simulink model "GuidanceLaw"  (R2023b)
settings: Solver=ode4  StartTime=0.0  StopTime=400  FixedStep=0.05  RelTol=1e-3
values from neighbouring files (symbols this model uses):
  APCMD_TYPE : value not decoded    [apDataDictionary.sldd]
  missionRoutePlan_struct = struct(      'validWpNum_u8', uint8(5),      'missionRoute_struct', repmat(wpDefault_struct, double(maxWpNum_u8), 1))    [initMissionRoutePlan_MC.m]
  MSSN_TYPE : value not decoded    [apDataDictionary.sldd]
  setPoint_struct = struct('lat_deg_d',double(31.200000),'lon_deg_d',double(121.500000),'alt_m_f',single(100),'yaw_deg_f',single(0))    [APTest.m]
undefined symbols (not defined in the file or in its folder): apParams
libraries: simulink x13, simulink_extras x3
(part 6 of 7)

== stateflow chart GuidanceLaw/Subsystem/TaskModeManager ==
  note: tryBwdTiltPlan函数完成其他条件的达成，包括规划是否成功
  state AUTO_BACKWARD_TILT
    entry:
    routeUpdate_b=candidateRouteUpdate_b;
    mssnType_u8=MSSN_TYPE.AUTO_BACKWARD_TILT;
    validWpNum_u8=candidateValidWpNum_u8;
    route_struct=candidateRoute_struct;
    during:
    routeUpdate_b=false;
  note: tryFwdTiltPlan函数完成其他条件的达成，包括规划是否成功
  state AUTO_FORWARD_TILT
    entry:
    routeUpdate_b=candidateRouteUpdate_b;
    mssnType_u8=MSSN_TYPE.AUTO_FORWARD_TILT;
    validWpNum_u8=candidateValidWpNum_u8;
    route_struct=candidateRoute_struct;
    during:
    routeUpdate_b=false;
  state ATT_EMERGENCY_LAND
    entry:
    routeUpdate_b=candidateRouteUpdate_b;
    mssnType_u8=mssnTypePre_u8;
    validWpNum_u8=candidateValidWpNum_u8;
    route_struct=candidateRoute_struct;
    during:
    routeUpdate_b=false;
  state IDLE
    entry:
    routeUpdate_b=false;
    mssnType_u8=MSSN_TYPE.IDLE;
    validWpNum_u8=uint8(0);
    route_struct=GenerateDefaultRoute();
  state RTH
    entry:
    routeUpdate_b=candidateRouteUpdate_b;
    mssnType_u8=MSSN_TYPE.RTH;
    validWpNum_u8=candidateValidWpNum_u8;
    route_struct=candidateRoute_struct;
    during:
    routeUpdate_b=false;
  state VERTICAL_TAKEOFF
    entry:
    routeUpdate_b=candidateRouteUpdate_b;
    mssnType_u8=MSSN_TYPE.VERTICAL_TAKEOFF;
    validWpNum_u8=candidateValidWpNum_u8;
    route_struct=candidateRoute_struct;
    during:
    routeUpdate_b=false;
  state ROUTE_FLIGHT
    entry:
    routeUpdate_b=candidateRouteUpdate_b;
    mssnType_u8=MSSN_TYPE.ROUTE_FLIGHT;
    validWpNum_u8=candidateValidWpNum_u8;
    route_struct=candidateRoute_struct;
    during:
    routeUpdate_b=false;
  state AUTO_LAND
    entry:
    note: 当前高度>盘旋最低高度，使用高度表高度？
    state AUTO_LAND_POINT_LOITER
      entry:
      routeUpdate_b=candidateRouteUpdate_b;
      mssnType_u8=MSSN_TYPE.AUTO_LAND_POINT_LOITER;
      validWpNum_u8=candidateValidWpNum_u8;
      route_struct=candidateRoute_struct;
      during:
      routeUpdate_b=false;
    state AUTO_LAND_DIRECTION_BACK_TILT
      entry:
      routeUpdate_b=candidateRouteUpdate_b;
      mssnType_u8=MSSN_TYPE.AUTO_LAND_DIRECTION_BACK_TILT;
      validWpNum_u8=candidateValidWpNum_u8;
      route_struct=candidateRoute_struct;
      during:
      routeUpdate_b=false;
    state AUTO_LAND_POINT_LAND
      entry:
      routeUpdate_b=candidateRouteUpdate_b;
      mssnType_u8=MSSN_TYPE.AUTO_LAND_POINT_LAND;
      validWpNum_u8=candidateValidWpNum_u8;
      route_struct=candidateRoute_struct;
      during:
      routeUpdate_b=false;
    state INVALID
      entry:
      routeUpdate_b = false;
      mssnType_u8 = mssnTypePre_u8;
      validWpNum_u8 = validWpNumPre_u8;
      route_struct = routePre_struct;
    (default) -> (junction 126)
    (junction 126) -> AUTO_LAND_POINT_LOITER [order 1] : [autoLandEntryType_u8 == uint8(1)]
    (junction 126) -> (junction 131) [order 2]
    INVALID -> AUTO_LAND_POINT_LOITER [order 3] : [autoLandEntryType_u8 == uint8(1)]
    AUTO_LAND_POINT_LOITER -> AUTO_LAND_DIRECTION_BACK_TILT : [(flightPhase_enum==FLIGHT_PHASE.TILT_FLIGHT || ...
        | flightPhase_enum==FLIGHT_PHASE.FW_FLIGHT) && ...
        | wpComplete_b && tryDirectionBackTiltPlan()]
    (junction 131) -> AUTO_LAND_DIRECTION_BACK_TILT [order 1] : [autoLandEntryType_u8 == uint8(2)]
    (junction 131) -> (junction 134) [order 2]
    INVALID -> AUTO_LAND_DIRECTION_BACK_TILT [order 2] : [autoLandEntryType_u8 == uint8(2)]
    AUTO_LAND_DIRECTION_BACK_TILT -> AUTO_LAND_POINT_LAND : [flightPhase_enum==FLIGHT_PHASE.MC_FLIGHT && tryPointLandPlan()]
    (junction 134) -> AUTO_LAND_POINT_LAND [order 1] : [autoLandEntryType_u8 == uint8(3)]
    (junction 134) -> INVALID [order 2]
    INVALID -> AUTO_LAND_POINT_LAND [order 1] : [autoLandEntryType_u8 == uint8(3)]
  (default) -> (junction 34)
  (junction 34) -> AUTO_BACKWARD_TILT [order 4] : [mssnTypePre_u8==MSSN_TYPE.AUTO_BACKWARD_TILT]{candidateRouteUpdate_b=false;...
      | candidateValidWpNum_u8=validWpNumPre_u8;candidateRoute_struct=routePre_struct}
  (junction 34) -> AUTO_FORWARD_TILT [order 5] : [mssnTypePre_u8==MSSN_TYPE.AUTO_FORWARD_TILT]{candidateRouteUpdate_b=false;...
      | candidateValidWpNum_u8=validWpNumPre_u8;candidateRoute_struct=routePre_struct}
  (junction 34) -> RTH [order 3] : [mssnTypePre_u8==MSSN_TYPE.RTH]{candidateRouteUpdate_b=false;...
      | candidateValidWpNum_u8=validWpNumPre_u8;candidateRoute_struct=routePre_struct}
  (junction 34) -> ROUTE_FLIGHT [order 2] : [mssnTypePre_u8==MSSN_TYPE.ROUTE_FLIGHT]{candidateRouteUpdate_b=false;...
      | candidateValidWpNum_u8=validWpNumPre_u8;candidateRoute_struct=routePre_struct}
  (junction 34) -> ATT_EMERGENCY_LAND [order 6] : [mssnTypePre_u8==MSSN_TYPE.ATT_LAND_ALTITUDE_LOITER || ...
      | mssnTypePre_u8==MSSN_TYPE.ATT_LAND_ATTITUDE_BACK_TILT ||...
      | mssnTypePre_u8==MSSN_TYPE.ATT_LAND_ATTITUDE_LAND]{candidateRouteUpdate_b=false;...
      | candidateValidWpNum_u8=validWpNumPre_u8;candidateRoute_struct=routePre_struct}
  (junction 34) -> VERTICAL_TAKEOFF [order 7] : [mssnTypePre_u8==MSSN_TYPE.VERTICAL_TAKEOFF]{candidateRouteUpdate_b=false;...
      | candidateValidWpNum_u8=validWpNumPre_u8;candidateRoute_struct=routePre_struct}
  (junction 34) -> AUTO_LAND [order 1] : [mssnTypePre_u8==MSSN_TYPE.AUTO_LAND_POINT_LOITER || ...
      | mssnTypePre_u8==MSSN_TYPE.AUTO_LAND_DIRECTION_BACK_TILT ||...
      | mssnTypePre_u8==MSSN_TYPE.AUTO_LAND_POINT_LAND]{candidateRouteUpdate_b=false;...
      | candidateValidWpNum_u8=validWpNumPre_u8;candidateRoute_struct=routePre_struct}
  (junction 34) -> IDLE [order 8]
  IDLE -> AUTO_FORWARD_TILT [order 1] : [flightPhase_enum==FLIGHT_PHASE.MC_FLIGHT && apTaskCmd_enum==AP_TASK_CMD.AUTO_FORWARD_TILT_CMD&&...
      | tryFwdTiltPlan()]
  IDLE -> AUTO_BACKWARD_TILT [order 2] : [flightPhase_enum==FLIGHT_PHASE.FW_FLIGHT && apTaskCmd_enum==AP_TASK_CMD.AUTO_BACKWARD_TILT_CMD&&...
      | tryBwdTiltPlan()]
  AUTO_BACKWARD_TILT -> IDLE : [ctrlLawApExec_b==false || apTaskCmd_enum==AP_TASK_CMD.AP_DISCONNECT_CMD||nonPilotCtrlSigFault_b==true]
  AUTO_FORWARD_TILT -> IDLE : [ctrlLawApExec_b==false || apTaskCmd_enum==AP_TASK_CMD.AP_DISCONNECT_CMD || ...
      | nonPilotCtrlSigFault_b==true]
  RTH -> IDLE [order 1] : [ctrlLawApExec_b==false || apTaskCmd_enum==AP_TASK_CMD.AP_DISCONNECT_CMD||nonPilotCtrlSigFault_b==true]
  ATT_EMERGENCY_LAND -> IDLE : [ctrlLawApExec_b==false || apTaskCmd_enum==AP_TASK_CMD.AP_DISCONNECT_CMD||nonPilotCtrlSigFault_b==true]
  IDLE -> RTH [order 3] : [(flightPhase_enum==FLIGHT_PHASE.MC_FLIGHT || ...
      | flightPhase_enum==FLIGHT_PHASE.TILT_FLIGHT || ...
      | flightPhase_enum==FLIGHT_PHASE.FW_FLIGHT) &&...
      | apTaskCmd_enum==AP_TASK_CMD.RTH_CMD && tryRTHPlan()]
  IDLE -> VERTICAL_TAKEOFF [order 4] : [flightPhase_enum==FLIGHT_PHASE.MC_GROUND && apTaskCmd_enum==AP_TASK_CMD.VERTICAL_TAKEOFF_CMD&&...
      | tryVerticalTakeoffPlan()]
  VERTICAL_TAKEOFF -> IDLE [order 1] : [ctrlLawApExec_b==false || apTaskCmd_enum==AP_TASK_CMD.AP_DISCONNECT_CMD||nonPilotCtrlSigFault_b==true]
  IDLE -> AUTO_LAND [order 6] : [(flightPhase_enum==FLIGHT_PHASE.MC_FLIGHT || ...
      | flightPhase_enum==FLIGHT_PHASE.TILT_FLIGHT || ...
      | flightPhase_enum==FLIGHT_PHASE.FW_FLIGHT ||...
      | flightPhase_enum==FLIGHT_PHASE.MC_GROUND) &&...
      | apTaskCmd_enum==AP_TASK_CMD.AUTO_LAND_CMD&&...
      | tryAutoLandPlan()]
  AUTO_LAND -> IDLE : [ctrlLawApExec_b==false || apTaskCmd_enum==AP_TASK_CMD.AP_DISCONNECT_CMD||nonPilotCtrlSigFault_b==true]
  ROUTE_FLIGHT -> IDLE [order 1] : [ctrlLawApExec_b==false || apTaskCmd_enum==AP_TASK_CMD.AP_DISCONNECT_CMD||nonPilotCtrlSigFault_b==true]
  IDLE -> ROUTE_FLIGHT [order 5] : [flightPhase_enum==FLIGHT_PHASE.MC_GROUND && apTaskCmd_enum==AP_TASK_CMD.ROUTE_FLIGHT_CMD && ...
      | tryRouteFlightPlan()]
  RTH -> AUTO_LAND [order 2] : [(flightPhase_enum==FLIGHT_PHASE.MC_FLIGHT || ...
      | flightPhase_enum==FLIGHT_PHASE.TILT_FLIGHT || ...
      | flightPhase_enum==FLIGHT_PHASE.FW_FLIGHT ||...
      | flightPhase_enum==FLIGHT_PHASE.MC_GROUND) &&...
      | apTaskCmd_enum==AP_TASK_CMD.AUTO_LAND_CMD&&...
      | tryAutoLandPlan()]
  ROUTE_FLIGHT -> RTH [order 3] : [(flightPhase_enum==FLIGHT_PHASE.MC_FLIGHT || ...
      | flightPhase_enum==FLIGHT_PHASE.TILT_FLIGHT || ...
      | flightPhase_enum==FLIGHT_PHASE.FW_FLIGHT) &&...
      | apTaskCmd_enum==AP_TASK_CMD.RTH_CMD && tryRTHPlan()]
  VERTICAL_TAKEOFF -> AUTO_LAND [order 2] : [(flightPhase_enum==FLIGHT_PHASE.MC_FLIGHT ||...
      | flightPhase_enum==FLIGHT_PHASE.MC_GROUND) &&...
      | apTaskCmd_enum==AP_TASK_CMD.AUTO_LAND_CMD &&...
      | tryAutoLandPlan()]
  ROUTE_FLIGHT -> AUTO_LAND [order 2] : [(flightPhase_enum==FLIGHT_PHASE.MC_FLIGHT || ...
      | flightPhase_enum==FLIGHT_PHASE.TILT_FLIGHT || ...
      | flightPhase_enum==FLIGHT_PHASE.FW_FLIGHT ||...
      | flightPhase_enum==FLIGHT_PHASE.MC_GROUND) &&...
      | apTaskCmd_enum==AP_TASK_CMD.AUTO_LAND_CMD&&...
      | tryAutoLandPlan()]
  data: planOk_b function_output; planOk_b function_output; planOk_b function_output; planOk_b function_output; planOk_b function_output; planOk_b function_output; planOk_b function_output; planOk_b function_output; planOk_b function_output; defaultRoute_struct function_output; planOk_b function_output; mssnType_u8 output Enum: MSSN_TYPE; routeUpdate_b output boolean; route_struct output Bus: wayPointBus size=[30 1]; flightPhase_enum input Enum: FLIGHT_PHASE; nav_struct input Bus: apTransNavBus; perfParams_struct input Bus: perfParamBus; ctrlLawApExec_b input boolean; apTaskCmd_enum input Enum: AP_TASK_CMD; faultInfo_struct input Bus: faultCaseBus; nonPilotCtrlSigFault_b input boolean; selectMssnModeParam input; candidateRoute_struct local Bus: wayPointBus size=[30 1]; candidateValidWpNum_u8 local uint8; mssnTypePre_u8 input Enum: MSSN_TYPE; routePre_struct input Bus: wayPointBus size=[30 1]; validWpNum_u8 output uint8; validWpNumPre_u8 input uint8; candidateRouteUpdate_b local boolean; fwdTiltPlanParam input; takeoffRltHgt_m_f input single; directBwdTiltPlanParam input; wpComplete_b input boolean; pointLoiterPlanParam input; pointLandParam input; missionRoutePlan_struct input; rthPoint_struct input; RTHParam input; bwdTiltPlanParam input; bwdTiltPoint_struct input; autoLandEntryType_u8 local uint8
  function planOk_b = tryFwdTiltPlan:
    | function planOk_b = tryFwdTiltPlan()
    | %#codegen
    | %
    | % 自动前倾航线规划
    | %
    | % 功能：
    | % 1. 根据当前水平地速方向或偏航角确定前倾方向；
    | % 2. 生成“当前点 -> 前倾方向点”两点航线；
    | % 3. 第一个航点为旋翼直线航点；
    | % 4. 第二个航点为固定翼直线航点。
    | 
    | %% 常量
    | degToRad_f = single(0.0174532925199433);
    | radToDeg_f = single(57.2957795130823);
    | zero_f = single(0.0);
    | 
    | planOk_b = false;
    | %% 计算前倾方向
    | velN_mps_f = nav_struct.velN_mps_f;
    | velE_mps_f = nav_struct.velE_mps_f;
    | yawCurrent_deg_f = cldWrap180(nav_struct.yaw_deg_f);
    | 
    | velNE_mps_f = sqrt(velN_mps_f * velN_mps_f + velE_mps_f * velE_mps_f);
    | 
    | if velNE_mps_f >= fwdTiltPlanParam(2)
    | 
    |     velCourse_deg_f = atan2(velE_mps_f, velN_mps_f) * radToDeg_f;
    |     velCourse_deg_f = cldWrap180(velCourse_deg_f);
    | 
    |     courseYawErr_deg_f = cldWrap180(velCourse_deg_f - yawCurrent_deg_f);
    | 
    |     courseYawLimit_deg_f = min(max(fwdTiltPlanParam(3), zero_f), single(180.0));
    | 
    |     if abs(courseYawErr_deg_f) <= courseYawLimit_deg_f
    |         fwdTiltYaw_deg_f = velCourse_deg_f;
    |     else
    |         return;
    |     end
    | else
    |     %% 默认使用当前偏航角
    |     fwdTiltYaw_deg_f = yawCurrent_deg_f;
    | end
    | 
    | %% 计算前倾方向点的水平偏移
    | 
    | fwdTiltYaw_rad_f = fwdTiltYaw_deg_f * degToRad_f;
    | 
    | offsetNorth_m_f = fwdTiltPlanParam(1) * cos(fwdTiltYaw_rad_f);
    | offsetEast_m_f = fwdTiltPlanParam(1) * sin(fwdTiltYaw_rad_f);
    | 
    | referenceLoc_deg_d = [nav_struct.lat_deg_d, nav_struct.lon_deg_d];
    | 
    | targetLoc_deg_d = offset(offsetNorth_m_f, offsetEast_m_f, referenceLoc_deg_d);
    | 
    | targetLat_deg_d = double(targetLoc_deg_d(1));
    | targetLon_deg_d = double(targetLoc_deg_d(2));
    | 
    | %% 初始化临时候选航线
    | 
    | routeTemp_struct = GenerateDefaultRoute();
    | 
    | %% 航点1：自动前倾起点
    | 
    | routeTemp_struct(1).wpType_u8 = WP_TYPE.MC_LINE_WP;
    | routeTemp_struct(1).lat_deg_d = nav_struct.lat_deg_d;
    | routeTemp_struct(1).lon_deg_d = nav_struct.lon_deg_d;
    | routeTemp_struct(1).alt_m_f = nav_struct.alt_m_f;
    | routeTemp_struct(1).spd_mps_f = zero_f;
    | routeTemp_struct(1).radius_m_f = zero_f;
    | routeTemp_struct(1).fastWp_b = true;
    | routeTemp_struct(1).yawType_u8 = uint8(1);
    | routeTemp_struct(1).yaw_deg_f = fwdTiltYaw_deg_f;
    | routeTemp_struct(1).timeOrCount_u16 = uint16(0);
    | routeTemp_struct(1).arrivalCond_u8 = uint8(0);
    | 
    | %% 航点2：固定翼方向航点
    | 
    | routeTemp_struct(2).wpType_u8 = WP_TYPE.FW_LINE_WP;
    | routeTemp_struct(2).lat_deg_d = targetLat_deg_d;
    | routeTemp_struct(2).lon_deg_d = targetLon_deg_d;
    | routeTemp_struct(2).alt_m_f = nav_struct.alt_m_f;
    | routeTemp_struct(2).spd_mps_f = fwdTiltPlanParam(4);    % 巡航速度
    | routeTemp_struct(2).radius_m_f = zero_f;
    | routeTemp_struct(2).fastWp_b = true;
    | routeTemp_struct(2).yawType_u8 = uint8(1);  % 航点指定
    | routeTemp_struct(2).yaw_deg_f = fwdTiltYaw_deg_f;
    | routeTemp_struct(2).timeOrCount_u16 = uint16(0);
    | routeTemp_struct(2).arrivalCond_u8 = uint8(0);
    | 
    | %% 规划成功后一次性提交候选航线
    | 
    | candidateRoute_struct = routeTemp_struct;
    | candidateValidWpNum_u8 = uint8(2);
    | candidateRouteUpdate_b = true;
    | planOk_b = candidateRouteUpdate_b;
    | 
    | end
  function planOk_b = tryRouteFlightPlan:
    | function planOk_b = tryRouteFlightPlan()
    | %#codegen
    | %
    | % 航线飞行规划
    | %
    | % 外部任务航线约定：
    | % 1. 外部航线只包含实际任务航点，不包含前航点锚点；
    | % 2. 外部首点必须是垂直起飞点；
    | % 3. 外部末点必须是垂直降落点。
    | %
    | % 内部规划航线：
    | % 1. 在首个垂直起飞点前增加当前位置起飞锚点；
    | % 2. 在末尾垂直降落点后增加一个垂直降落执行点；
    | % 3. 形成：
    | %       MC_TAKEOFF_WP -> MC_TAKEOFF_WP
    | %       MC_LAND_WP    -> MC_LAND_WP
    | 
    | routeTemp_struct = GenerateDefaultRoute();
    | 
    | planOk_b = false;
    | 
    | maxWpNum_u8 = uint8(numel(routeTemp_struct));
    | missionValidWpNumTemp_u8 = missionRoutePlan_struct.validWpNum_u8;
    | mssnRoute_struct = missionRoutePlan_struct.missionRoute_struct;
    | %% 检查外部任务航点数量
    | 
    | % 至少包含：
    | % 1. 垂直起飞目标点；
    | % 2. 垂直降落点。
    | %
    | % 内部规划还需要增加：
    | % 1. 起飞锚点；
    | % 2. 垂直降落执行点。
    | if missionValidWpNumTemp_u8 < uint8(2)
    |     return;
    | end
    | 
    | if missionValidWpNumTemp_u8 > maxWpNum_u8 - uint8(2)
    |     return;
    | end
    | 
    | %% 检查外部航线首尾结构
    | fpMssnRoute_struct = mssnRoute_struct(1);
    | if fpMssnRoute_struct.wpType_u8 ~= WP_TYPE.MC_TAKEOFF_WP
    |     return;
    | end
    | 
    | epMssnRoute_struct = mssnRoute_struct(missionValidWpNumTemp_u8);
    | if epMssnRoute_struct.wpType_u8 ~= WP_TYPE.MC_LAND_WP
    |     return;
    | end
    | 
    | %% 计算内部航线有效点数
    | 
    | validWpNumTemp_u8 = missionValidWpNumTemp_u8 + uint8(2);
    | 
    | %% 将外部任务航线复制到内部航线第2点开始的位置
    | 
    | % 内部第1点留给起飞锚点。
    | for missionWpIdx_u8 = uint8(1):missionValidWpNumTemp_u8
    | 
    |     routeWpIdx_u8 = missionWpIdx_u8 + uint8(1);
    | 
    |     routeTemp_struct(routeWpIdx_u8) = mssnRoute_struct(missionWpIdx_u8);
    | 
    | end
    | 
    | %% 增加垂直起飞前航点锚点
    | 
    | routeTemp_struct(1) = routeTemp_struct(2);
    | 
    | routeTemp_struct(1).wpType_u8 = WP_TYPE.MC_TAKEOFF_WP;
    | routeTemp_struct(1).lat_deg_d = nav_struct.lat_deg_d;
    | routeTemp_struct(1).lon_deg_d = nav_struct.lon_deg_d;
    | routeTemp_struct(1).alt_m_f = nav_struct.alt_m_f;
    | routeTemp_struct(1).spd_mps_f = single(0.0);
    | routeTemp_struct(1).radius_m_f = single(0.0);
    | routeTemp_struct(1).fastWp_b = false;
    | routeTemp_struct(1).yawType_u8 = uint8(0);      % 起飞时锁定当前偏航角，用不到这个标志
    | routeTemp_struct(1).yaw_deg_f = nav_struct.yaw_deg_f;
    | routeTemp_struct(1).timeOrCount_u16 = uint16(0);
    | routeTemp_struct(1).arrivalCond_u8 = uint8(0);
    | 
    | %% 增加垂直降落执行点
    | 
    | % 两个点使用相同水平位置、高度和航向，避免航段切换时发生水平位置、目标高度或偏航角跳变。
    | % 垂直降落过程根据相对地面高度生成下降指令，不依赖此处接地点高度。
    | 
    | landEntryWpIdx_u8 = validWpNumTemp_u8 - uint8(1);
    | landExecWpIdx_u8 = validWpNumTemp_u8;
    | 
    | routeTemp_struct(landExecWpIdx_u8) = routeTemp_struct(landEntryWpIdx_u8);
    | 
    | routeTemp_struct(landExecWpIdx_u8).wpType_u8 = WP_TYPE.MC_LAND_WP;
    | routeTemp_struct(landExecWpIdx_u8).spd_mps_f = single(0.0);
    | routeTemp_struct(landExecWpIdx_u8).radius_m_f = single(0.0);
    | routeTemp_struct(landExecWpIdx_u8).fastWp_b = false;
    | routeTemp_struct(landExecWpIdx_u8).timeOrCount_u16 = uint16(0);
    | routeTemp_struct(landExecWpIdx_u8).arrivalCond_u8 = uint8(0);
    | 
    | %% 检查内部实际执行航段组合
    | 
    | routeValid_b = true;
    | curWpIdxTemp_u8 = uint8(2);
    | 
    | % 每次循环至少推进一个航点，因此最大循环次数不超过航线容量。
    | for checkCnt_u8 = uint8(1):maxWpNum_u8
    | 
    |     if routeValid_b && curWpIdxTemp_u8 <= validWpNumTemp_u8
    | 
    |         preWpType_u8 = routeTemp_struct(curWpIdxTemp_u8 - uint8(1)).wpType_u8;
    |         curWpType_u8 = routeTemp_struct(curWpIdxTemp_u8).wpType_u8;
    | 
    |         pairValid_b = false;
    | 
    |         %% 垂直起飞航点
    | 
    |         % 内部航线只允许第2点为垂直起飞目标点。
    |         % 第1点和第2点必须同时为垂直起飞航点。
    |         if curWpType_u8 == WP_TYPE.MC_TAKEOFF_WP
    | 
    |             pairValid_b = curWpIdxTemp_u8 == uint8(2) && preWpType_u8 == WP_TYPE.MC_TAKEOFF_WP;
    | 
    |         %% 垂直降落航点
    | 
    |         elseif curWpType_u8 == WP_TYPE.MC_LAND_WP
    | 
    |             if preWpType_u8 == WP_TYPE.MC_LAND_WP
    | 
    |                 % MC_LAND_WP -> MC_LAND_WP为垂直降落航段。
    |                 % 第二个垂直降落点必须是整条航线最后一点。
    |                 pairValid_b = curWpIdxTemp_u8 == validWpNumTemp_u8;
    | 
    |             else
    | 
    |                 landEntryPreValid_b = preWpType_u8 == WP_TYPE.MC_TAKEOFF_WP || preWpType_u8 == WP_TYPE.MC_LINE_WP || preWpType_u8 == WP_TYPE.FW_LINE_WP;
    | 
    |                 % 第一个垂直降落点必须是倒数第2点，
    |                 % 后面必须紧跟垂直降落执行点。
    |                 landPairComplete_b = curWpIdxTemp_u8 + uint8(1) == validWpNumTemp_u8;
    | 
    |                 if landPairComplete_b
    |                     landPairComplete_b = routeTemp_struct(curWpIdxTemp_u8 + uint8(1)).wpType_u8 == WP_TYPE.MC_LAND_WP;
    |                 end
    | 
    |                 pairValid_b = landEntryPreValid_b && landPairComplete_b;
    | 
    |             end
    | 
    |         %% 旋翼直线航点
    | 
    |         elseif curWpType_u8 == WP_TYPE.MC_LINE_WP
    | 
    |             pairValid_b = preWpType_u8 == WP_TYPE.MC_TAKEOFF_WP || preWpType_u8 == WP_TYPE.MC_LINE_WP || preWpType_u8 == WP_TYPE.FW_LINE_WP;
    | 
    |         %% 固定翼直线航点
    | 
    |         elseif curWpType_u8 == WP_TYPE.FW_LINE_WP
    | 
    |             pairValid_b = preWpType_u8 == WP_TYPE.MC_TAKEOFF_WP || preWpType_u8 == WP_TYPE.MC_LINE_WP || preWpType_u8 == WP_TYPE.FW_LINE_WP;
    | 
    |         %% 固定翼圆弧航点
    | 
    |         elseif curWpType_u8 == WP_TYPE.FW_CIR_WP
    | 
    |             pairValid_b = preWpType_u8 == WP_TYPE.FW_LINE_WP;
    | 
    |         end
    | 
    |         if ~pairValid_b
    | 
    |             routeValid_b = false;
    | 
    |         elseif curWpType_u8 == WP_TYPE.FW_CIR_WP
    | 
    |             %% 检查固定翼圆弧切出结构
    | 
    |             % 圆弧航点后必须依次存在：
    |             % 1. 固定翼直线切出辅助点；
    |             % 2. 圆弧退出后真正执行的目标点。
    |             if curWpIdxTemp_u8 + uint8(2) > validWpNumTemp_u8
    | 
    |                 routeValid_b = false;
    | 
    |             elseif routeTemp_struct(curWpIdxTemp_u8 + uint8(1)).wpType_u8 ~= WP_TYPE.FW_LINE_WP
    | 
    |                 routeValid_b = false;
    | 
    |             else
    | 
    |                 % 跳过圆弧切出辅助点。
    |                 curWpIdxTemp_u8 = curWpIdxTemp_u8 + uint8(2);
    | 
    |             end
    | 
    |         else
    | 
    |             curWpIdxTemp_u8 = curWpIdxTemp_u8 + uint8(1);
    | 
    |         end
    | 
    |     end
    | 
    | end
    | 
    | %% 检查是否完成全部有效航点遍历
    | 
    | if ~routeValid_b || curWpIdxTemp_u8 <= validWpNumTemp_u8
    |     return;
    | end
    | 
    | %% 原子更新候选航线
    | 
    | candidateRoute_struct = routeTemp_struct;
    | candidateValidWpNum_u8 = validWpNumTemp_u8;
    | candidateRouteUpdate_b = true;
    | 
    | planOk_b = true;
    | 
    | end
  function planOk_b = tryBwdTiltPlan:
    | function planOk_b = tryBwdTiltPlan()
    | %#codegen
    | %
    | % 自动后倾航线规划
    | %
    | % 功能：
    | % 1. 判断飞机是否处于自动后倾允许高度范围；
    | % 2. 判断当前速度方向是否指向预设后倾点；
    | % 3. 判断当前位置是否位于后倾点的进场方向范围内；
    | % 4. 根据后倾速度导引计算动态减速捕获区；
    | % 5. 飞机进入捕获区后生成FW_LINE_WP -> MC_LINE_WP航线；
    | % 6. 固定翼/倾转阶段沿航线减速后倾，进入旋翼阶段后继续飞向后倾点并减速悬停。
    | 
    | planOk_b = false;
    | 
    | zero_f = single(0.0);
    | radToDeg_f = single(57.29577951308232);
    | minPathLength_m_f = single(1.0);
    | 
    | %% 参数解析
    | 
    | minBackTiltHag_m_f = max(single(bwdTiltPlanParam(1)), zero_f);
    | 
    | maxBackTiltHag_m_f = max(single(bwdTiltPlanParam(2)), minBackTiltHag_m_f);
    | 
    | velocityCaptureAngle_deg_f = min(max(single(bwdTiltPlanParam(3)), zero_f), single(180.0));
    | 
    | approachCaptureAngle_deg_f = min(max(single(bwdTiltPlanParam(4)), zero_f), single(180.0));
    | 
    | captureLeadTime_s_f = max(single(bwdTiltPlanParam(5)), zero_f);
    | 
    | % 与fwAirSpdGuidance中的保护方式保持一致
    | backTransDecel_mps2_f = max(single(bwdTiltPlanParam(6)), single(0.1));
    | 
    | backTransStopRadius_m_f = max(single(bwdTiltPlanParam(7)), zero_f);
    | 
    | %% 检查相对高度
    | 
    | % if ~nav_struct.hagValid_b
    | %     return;
    | % end
    | 
    | currentHag_m_f = single(nav_struct.hag_m_f);
    | 
    | if currentHag_m_f < minBackTiltHag_m_f || currentHag_m_f > maxBackTiltHag_m_f
    |     return;
    | end
    | 
    | %% 计算当前水平地速
    | 
    | velN_mps_f = single(nav_struct.velN_mps_f);
    | velE_mps_f = single(nav_struct.velE_mps_f);
    | 
    | groundSpdSq_m2ps2_f = velN_mps_f * velN_mps_f + velE_mps_f * velE_mps_f;
    | 
    | groundSpd_mps_f = sqrt(max(groundSpdSq_m2ps2_f, zero_f));
    | 
    | % if groundSpd_mps_f < single(5)
    | %     return;
    | % end
    | 
    | %% 计算当前位置到后倾点的NE向量
    | 
    | currentLoc_deg_d = [nav_struct.lat_deg_d, nav_struct.lon_deg_d];
    | 
    | backTiltLoc_deg_d = [bwdTiltPoint_struct.lat_deg_d, bwdTiltPoint_struct.lon_deg_d];
    | 
    | targetVectorNE_m_f = getDistanceNE(currentLoc_deg_d, backTiltLoc_deg_d);
    | 
    | targetVectorN_m_f = targetVectorNE_m_f(1);
    | targetVectorE_m_f = targetVectorNE_m_f(2);
    | 
    | targetDistSq_m2_f = targetVectorN_m_f * targetVectorN_m_f + targetVectorE_m_f * targetVectorE_m_f;
    | 
    | targetDist_m_f = sqrt(max(targetDistSq_m2_f, zero_f));
    | 
    | if targetDist_m_f < minPathLength_m_f
    |     return;
    | end
    | 
    | %% 计算速度方向和目标方向
    | 
    | velocityCourse_deg_f = atan2(velE_mps_f, velN_mps_f) * radToDeg_f;
    | 
    | velocityCourse_deg_f = cldWrap180(velocityCourse_deg_f);
    | 
    | targetBearing_deg_f = atan2(targetVectorE_m_f, targetVectorN_m_f) * radToDeg_f;
    | 
    | targetBearing_deg_f = cldWrap180(targetBearing_deg_f);
    | 
    | %% 检查速度方向捕获条件
    | 
    | velocityTargetErr_deg_f = cldWrap180(velocityCourse_deg_f - targetBearing_deg_f);
    | 
    | if abs(velocityTargetErr_deg_f) > velocityCaptureAngle_deg_f
    |     return;
    | end
    | 
    | %% 检查预设进场方向
    | 
    | approachHdg_deg_f = cldWrap180(single(bwdTiltPoint_struct.yaw_deg_f));
    | 
    | approachErr_deg_f = cldWrap180(targetBearing_deg_f - approachHdg_deg_f);
    | 
    | if abs(approachErr_deg_f) > approachCaptureAngle_deg_f
    |     return;
    | end
    | 
    | %% 根据后倾速度包线计算动态捕获距离
    | 
    | % 当前自动后倾最终需要在后倾点悬停，虚拟末速度为0。
    | backTiltFinalSpd_mps_f = zero_f;
    | 
    | speedDiffSq_m2ps2_f = groundSpd_mps_f * groundSpd_mps_f - backTiltFinalSpd_mps_f * backTiltFinalSpd_mps_f;
    | 
    | speedDiffSq_m2ps2_f = max(speedDiffSq_m2ps2_f, zero_f);
    | 
    | brakeDist_m_f = speedDiffSq_m2ps2_f / (single(2.0) * backTransDecel_mps2_f);
    | 
    | idealCaptureDist_m_f = backTransStopRadius_m_f + brakeDist_m_f;
    | 
    | % 允许提前一小段时间进入自动后倾状态。
    | captureLeadDist_m_f = groundSpd_mps_f * captureLeadTime_s_f;
    | 
    | maxCaptureDist_m_f = idealCaptureDist_m_f + captureLeadDist_m_f;
    | 
    | %% 检查动态距离捕获区
    | 
    | % 距离过短时，现有速度导引无法按照设定减速度停在后倾点。
    | if targetDist_m_f < idealCaptureDist_m_f
    |     return;
    | end
    | 
    | % 距离过远时暂不进入自动后倾，等待飞机继续接近后倾点。
    | if targetDist_m_f > maxCaptureDist_m_f
    |     return;
    | end
    | 
    | %% 初始化候选航线
    | 
    | routeTemp_struct = GenerateDefaultRoute();
    | 
    | %% W1：自动后倾起始锚点
    | 
    | routeTemp_struct(1).wpType_u8 = WP_TYPE.FW_LINE_WP;
    | routeTemp_struct(1).lat_deg_d = nav_struct.lat_deg_d;
    | routeTemp_struct(1).lon_deg_d = nav_struct.lon_deg_d;
    | routeTemp_struct(1).alt_m_f = nav_struct.alt_m_f;
    | routeTemp_struct(1).spd_mps_f = groundSpd_mps_f;
    | routeTemp_struct(1).radius_m_f = zero_f;
    | routeTemp_struct(1).fastWp_b = false;
    | routeTemp_struct(1).yawType_u8 = uint8(1);
    | routeTemp_struct(1).yaw_deg_f = approachHdg_deg_f;
    | routeTemp_struct(1).timeOrCount_u16 = uint16(0);
    | routeTemp_struct(1).arrivalCond_u8 = uint8(0);
    | 
    | %% W2：预设自动后倾点
    | 
    | routeTemp_struct(2).wpType_u8 = WP_TYPE.MC_LINE_WP;
    | routeTemp_struct(2).lat_deg_d = bwdTiltPoint_struct.lat_deg_d;
    | routeTemp_struct(2).lon_deg_d = bwdTiltPoint_struct.lon_deg_d;
    | 
    | % 自动后倾只完成构型转换和水平减速，转换期间保持当前高度。
    | routeTemp_struct(2).alt_m_f = nav_struct.alt_m_f;
    | 
    | routeTemp_struct(2).spd_mps_f = zero_f;
    | routeTemp_struct(2).radius_m_f = zero_f;
    | 
    | % false使后倾速度导引采用零虚拟末速度。
    | routeTemp_struct(2).fastWp_b = false;
    | 
    | % 旋翼阶段减速过程中保持设定进场航向。
    | routeTemp_struct(2).yawType_u8 = uint8(1);      % 航点指定
    | routeTemp_struct(2).yaw_deg_f = approachHdg_deg_f;
    | routeTemp_struct(2).timeOrCount_u16 = uint16(0);
    | routeTemp_struct(2).arrivalCond_u8 = uint8(0);
    | 
    | %% 提交候选航线
    | 
    | candidateRoute_struct = routeTemp_struct;
    | candidateValidWpNum_u8 = uint8(2);
    | candidateRouteUpdate_b = true;
    | 
    | planOk_b = true;
    | 
    | end
  function planOk_b = tryAutoLandPointLoiterPlan:
    | function planOk_b = tryAutoLandPointLoiterPlan()
    | %#codegen
    | %
    | % 自动着陆定点盘旋降高航线规划
    | %
    | % 高度选择：
    | % 1. hagValid_b为true时，使用实测HAG；
    | % 2. hagValid_b为false时，使用当前绝对高度减去Home点地面绝对高度。
    | %
    | % rthPoint_struct.alt_m_f：
    | % Home点地面绝对高度，必须与nav_struct.alt_m_f使用相同高度基准。
    | %
    | % pointLoiterPlanParam：
    | % 1：进入盘旋的高度裕度，m，应不小于圆弧高度到达容差；
    | % 2：重力加速度，m/s^2；
    | % 3：最小盘旋半径，m。
    | 
    | planOk_b = false;
    | 
    | zero_f = single(0.0);
    | minGroundSpd_mps_f = single(0.1);
    | loiterRollUseRatio_f = single(0.8);
    | minTanRoll_f = single(1.0e-3);
    | 
    | %% 参数读取
    | 
    | loiterEntryMargin_m_f = max(single(pointLoiterPlanParam(1)), zero_f);
    | G_mps2_f = single(pointLoiterPlanParam(2));
    | minLoiterRadius_m_f = max(single(pointLoiterPlanParam(3)), zero_f);
    | 
    | backTiltTargetHag_m_f = max(single(selectMssnModeParam(2)), zero_f);
    | 
    | currentAlt_m_f = single(nav_struct.alt_m_f);
    | 
    | %% 选择地面高度基准并计算规划用离地高度
    | 
    | if nav_struct.hagValid_b
    | 
    |     % HAG有效：使用实测HAG。
    |     hagForPlan_m_f = max(single(nav_struct.hag_m_f), zero_f);
    | 
    |     % 由同一时刻的绝对高度和HAG反算当前位置地面绝对高度。
    |     groundAltForPlan_m_f = currentAlt_m_f - hagForPlan_m_f;
    | 
    | else
    | 
    |     % HAG无效：使用Home点地面绝对高度。
    |     groundAltForPlan_m_f = single(rthPoint_struct.alt_m_f);
    | 
    |     hagForPlan_m_f = currentAlt_m_f - groundAltForPlan_m_f;
    | 
    |     % 防止高度基准配置误差产生负离地高度。
    |     hagForPlan_m_f = max(hagForPlan_m_f, zero_f);
    | 
    | end
    | 
    | 
    | %% 判断是否需要盘旋降高
    | 
    | loiterEntryHag_m_f = backTiltTargetHag_m_f + loiterEntryMargin_m_f;
    | 
    | % 已经进入允许直接定向后倾的高度范围，不生成盘旋航线。
    | if hagForPlan_m_f <= loiterEntryHag_m_f
    |     return;
    | end
    | 
    | %% 计算定向后倾目标绝对高度
    | 
    | backTiltTargetAlt_m_f = groundAltForPlan_m_f + backTiltTargetHag_m_f;
    | 
    | %% 计算当前水平地速
    | 
    | velN_mps_f = single(nav_struct.velN_mps_f);
    | velE_mps_f = single(nav_struct.velE_mps_f);
    | 
    | groundSpdSq_m2ps2_f = velN_mps_f * velN_mps_f + velE_mps_f * velE_mps_f;
    | groundSpd_mps_f = sqrt(max(groundSpdSq_m2ps2_f, zero_f));
    | 
    | if groundSpd_mps_f < minGroundSpd_mps_f
    |     return;
    | end
    | 
    | unitVelN_f = velN_mps_f / groundSpd_mps_f;
    | unitVelE_f = velE_mps_f / groundSpd_mps_f;
    | 
    | loiterSpd_mps_f = groundSpd_mps_f;
    | 
    | %% 根据当前滚转方向选择盘旋方向
    | 
    | if nav_struct.roll_deg_f >= zero_f
    |     loiterDirection_f = single(1.0);
    | else
    |     loiterDirection_f = single(-1.0);
    | end
    | 
    | %% 计算可用盘旋滚转角
    | 
    | if loiterDirection_f > zero_f
    |     availableRoll_deg_f = max(abs(perfParams_struct.maxRollAngle_deg_f), zero_f);
    | else
    |     availableRoll_deg_f = max(abs(perfParams_struct.minRollAngle_deg_f), zero_f);
    | end
    | 
    | loiterRoll_deg_f = availableRoll_deg_f * loiterRollUseRatio_f;
    | loiterRoll_rad_f = loiterRoll_deg_f * single(pi / 180.0);
    | 
    | tanLoiterRoll_f = max(tan(loiterRoll_rad_f), minTanRoll_f);
    | 
    | % if tanLoiterRoll_f <= minTanRoll_f
    | %     return;
    | % end
    | 
    | %% 计算盘旋半径
    | 
    | turnRadiusRaw_m_f = groundSpdSq_m2ps2_f / (G_mps2_f * tanLoiterRoll_f);
    | turnRadius_m_f = max(turnRadiusRaw_m_f, minLoiterRadius_m_f);
    | 
    | %% 计算盘旋圆心
    | 
    | centerOffsetN_m_f = -loiterDirection_f * unitVelE_f * turnRadius_m_f;
    | centerOffsetE_m_f = loiterDirection_f * unitVelN_f * turnRadius_m_f;
    | 
    | referenceLL_deg_d = [nav_struct.lat_deg_d, nav_struct.lon_deg_d];
    | 
    | centerLL_deg_d = offset(centerOffsetN_m_f, centerOffsetE_m_f, referenceLL_deg_d);
    | 
    | signedRadius_m_f = loiterDirection_f * turnRadius_m_f;
    | 
    | %% 生成盘旋航线
    | 
    | routeTemp_struct = GenerateDefaultRoute();
    | 
    | %% 1号点：当前位置锚点
    | 
    | routeTemp_struct(1).wpType_u8 = WP_TYPE.FW_LINE_WP;
    | routeTemp_struct(1).lat_deg_d = nav_struct.lat_deg_d;
    | routeTemp_struct(1).lon_deg_d = nav_struct.lon_deg_d;
    | routeTemp_struct(1).alt_m_f = currentAlt_m_f;
    | routeTemp_struct(1).spd_mps_f = loiterSpd_mps_f;
    | routeTemp_struct(1).radius_m_f = zero_f;
    | routeTemp_struct(1).fastWp_b = false;
    | routeTemp_struct(1).yawType_u8 = uint8(0);
    | routeTemp_struct(1).yaw_deg_f = nav_struct.yaw_deg_f;
    | routeTemp_struct(1).timeOrCount_u16 = uint16(0);
    | routeTemp_struct(1).arrivalCond_u8 = uint8(0);
    | 
    | %% 2号点：盘旋圆心
    | 
    | routeTemp_struct(2).wpType_u8 = WP_TYPE.FW_CIR_WP;
    | routeTemp_struct(2).lat_deg_d = centerLL_deg_d(1);
    | routeTemp_struct(2).lon_deg_d = centerLL_deg_d(2);
    | routeTemp_struct(2).alt_m_f = backTiltTargetAlt_m_f;
    | routeTemp_struct(2).spd_mps_f = loiterSpd_mps_f;
    | routeTemp_struct(2).radius_m_f = signedRadius_m_f;
    | routeTemp_struct(2).fastWp_b = false;
    | routeTemp_struct(2).yawType_u8 = uint8(0);
    | routeTemp_struct(2).yaw_deg_f = nav_struct.yaw_deg_f;
    | routeTemp_struct(2).timeOrCount_u16 = uint16(0);
    | 
    | % 高度和切出方位角同时满足后完成圆弧。
    | routeTemp_struct(2).arrivalCond_u8 = uint8(3);
    | 
    | %% 3号点：圆弧切出点
    | 
    | routeTemp_struct(3).wpType_u8 = WP_TYPE.FW_LINE_WP;
    | routeTemp_struct(3).lat_deg_d = nav_struct.lat_deg_d;
    | routeTemp_struct(3).lon_deg_d = nav_struct.lon_deg_d;
    | routeTemp_struct(3).alt_m_f = backTiltTargetAlt_m_f;
    | routeTemp_struct(3).spd_mps_f = loiterSpd_mps_f;
    | routeTemp_struct(3).radius_m_f = zero_f;
    | routeTemp_struct(3).fastWp_b = false;
    | routeTemp_struct(3).yawType_u8 = uint8(0);
    | routeTemp_struct(3).yaw_deg_f = nav_struct.yaw_deg_f;
    | routeTemp_struct(3).timeOrCount_u16 = uint16(0);
    | routeTemp_struct(3).arrivalCond_u8 = uint8(0);
    | 
    | %% 提交候选航线
    | 
    | candidateRoute_struct = routeTemp_struct;
    | candidateValidWpNum_u8 = uint8(3);
    | candidateRouteUpdate_b = true;
    | 
    | planOk_b = true;
    | 
    | end
  function planOk_b = tryAutoLandPointLoiterPlan1:
    | function planOk_b = tryAutoLandPointLoiterPlan1
    | %#codegen
    | %
    | % 自动着陆定点盘旋降高航线规划
    | %
    | % 1号点：进入盘旋时的当前位置锚点
    | % 2号点：盘旋圆心，目标高度为定向后倾高度，使用arrivalCond_u8=3，即“高度+方位角”。
    | % 3号点：圆弧切出点，水平位置与进入点相同
    | 
    | %% 必要条件
    | 
    | G_mps2_f = pointLoiterPlanParam(2);
    | minLoiterHgt_m_f = max(single(selectMssnModeParam(2)), single(0.0));
    | minLoiterRadius_m_f = pointLoiterPlanParam(3);
    | 
    | %% 计算盘旋速度
    | 
    | velN_mps_f = single(nav_struct.velN_mps_f);
    | velE_mps_f = single(nav_struct.velE_mps_f);
    | 
    | groundSpd_mps_f = sqrt(velN_mps_f * velN_mps_f + velE_mps_f * velE_mps_f);
    | 
    | % loiterSpd_mps_f = max(max(single(loiterSpdPlan_mps_f), single(0.0)), groundSpd_mps_f);
    | loiterSpd_mps_f = max(single(0.0), groundSpd_mps_f);
    | 
    | unitVelN_f = velN_mps_f / groundSpd_mps_f;
    | unitVelE_f = velE_mps_f / groundSpd_mps_f;
    | 
    | %% 确定盘旋方向
    | 
    | if nav_struct.roll_deg_f >= single(0)
    |     loiterDirection_f = single(1.0);        %NE坐标系中的N轴向E轴转动方向
    | else
    |     loiterDirection_f = single(-1.0);
    | end
    | 
    | %% 确定有效盘旋滚转角
    | 
    | if loiterDirection_f > single(0.0)
    |     availableRoll_deg_f = max(abs(perfParams_struct.maxRollAngle_deg_f), single(0.0));
    | else
    |     availableRoll_deg_f = max(abs(perfParams_struct.minRollAngle_deg_f), single(0.0));
    | end
    | 
    | %% 计算盘旋半径
    | 
    | loiterRoll_rad_f = availableRoll_deg_f * single(pi / 180.0) * single(0.8);    % 直接按照极限角度计算的半径？*0.8？
    | 
    | tan_loiterRoll_rad_f = max(tan(loiterRoll_rad_f),single(1e-2));     % 除零保护
    | 
    | turnRadiusRaw_m_f = loiterSpd_mps_f * loiterSpd_mps_f / (G_mps2_f * tan_loiterRoll_rad_f);
    | 
    | turnRadius_m_f = max(turnRadiusRaw_m_f, max(single(minLoiterRadius_m_f), single(0.0)));
    | 
    | %% 计算盘旋圆心
    | 
    | centerOffsetN_m_f = -loiterDirection_f * unitVelE_f * turnRadius_m_f;
    | centerOffsetE_m_f =  loiterDirection_f * unitVelN_f * turnRadius_m_f;
    | 
    | referenceLL_deg_d = [nav_struct.lat_deg_d, nav_struct.lon_deg_d];
    | 
    | centerLL_deg_d = offset(centerOffsetN_m_f, centerOffsetE_m_f, referenceLL_deg_d);
    | 
    | signedRadius_m_f = loiterDirection_f * turnRadius_m_f;
    | 
    | %% 计算盘旋目标绝对高度
    | 
    | groundAlt_m_f = single(nav_struct.alt_m_f) - single(nav_struct.hag_m_f);
    | minLoiterAlt_m_f = groundAlt_m_f + minLoiterHgt_m_f;
    | 
    | %% 生成盘旋航线
    | 
    | routeTemp_struct = GenerateDefaultRoute();
    | 
    | % 1号点：当前位置锚点
    | 
    | routeTemp_struct(1).wpType_u8 = WP_TYPE.FW_LINE_WP;
    | routeTemp_struct(1).lat_deg_d = nav_struct.lat_deg_d;
    | routeTemp_struct(1).lon_deg_d = nav_struct.lon_deg_d;
    | routeTemp_struct(1).alt_m_f = nav_struct.alt_m_f;
    | routeTemp_struct(1).spd_mps_f = loiterSpd_mps_f;
    | routeTemp_struct(1).radius_m_f = single(0.0);
    | routeTemp_struct(1).fastWp_b = false;
    | routeTemp_struct(1).yawType_u8 = uint8(0);
    | routeTemp_struct(1).yaw_deg_f = nav_struct.yaw_deg_f;
    | routeTemp_struct(1).timeOrCount_u16 = uint16(0);
    | routeTemp_struct(1).arrivalCond_u8 = uint8(0);
    | 
    | % 2号点：盘旋圆心
    | 
    | routeTemp_struct(2).wpType_u8 = WP_TYPE.FW_CIR_WP;
    | routeTemp_struct(2).lat_deg_d = centerLL_deg_d(1);
    | routeTemp_struct(2).lon_deg_d = centerLL_deg_d(2);
    | routeTemp_struct(2).alt_m_f = minLoiterAlt_m_f;
    | routeTemp_struct(2).spd_mps_f = loiterSpd_mps_f;
    | routeTemp_struct(2).radius_m_f = signedRadius_m_f;
    | routeTemp_struct(2).fastWp_b = false;
    | routeTemp_struct(2).yawType_u8 = uint8(0);
    | routeTemp_struct(2).yaw_deg_f = nav_struct.yaw_deg_f;
    | routeTemp_struct(2).timeOrCount_u16 = uint16(0);
    | routeTemp_struct(2).arrivalCond_u8 = uint8(3);          % 方位角+海拔高度判定条件
    | 
    | % 3号点：圆弧切出点
    | 
    | routeTemp_struct(3).wpType_u8 = WP_TYPE.FW_LINE_WP;
    | routeTemp_struct(3).lat_deg_d = nav_struct.lat_deg_d;
    | routeTemp_struct(3).lon_deg_d = nav_struct.lon_deg_d;
    | routeTemp_struct(3).alt_m_f = minLoiterAlt_m_f;
    | routeTemp_struct(3).spd_mps_f = loiterSpd_mps_f;
    | routeTemp_struct(3).radius_m_f = single(0.0);
    | routeTemp_struct(3).fastWp_b = false;
    | routeTemp_struct(3).yawType_u8 = uint8(0);
    | routeTemp_struct(3).yaw_deg_f = nav_struct.yaw_deg_f;
    | routeTemp_struct(3).timeOrCount_u16 = uint16(0);
    | routeTemp_struct(3).arrivalCond_u8 = uint8(0);
    | 
    | %% 提交候选航线
    | 
    | candidateRoute_struct = routeTemp_struct;
    | candidateValidWpNum_u8 = uint8(3);
    | candidateRouteUpdate_b = true;
    | 
    | planOk_b = candidateRouteUpdate_b;
    | 
    | end
  function planOk_b = tryRTHPlan:
    | function planOk_b = tryRTHPlan()
    | %#codegen
    | %
    | %% 调用返航规划器
    | 
    | [routeTemp_struct, validNum_u8, routePlanValid_b] = returnPlan(rthPoint_struct, flightPhase_enum, RTHParam, perfParams_struct, ...
    |     pointLandParam, nav_struct);
    | 
    | %% 规划成功后一次性提交候选航线
    | 
    | candidateRoute_struct = routeTemp_struct;
    | candidateValidWpNum_u8 = validNum_u8;
    | candidateRouteUpdate_b = routePlanValid_b;
    | 
    | planOk_b = candidateRouteUpdate_b;
    | end
  function planOk_b = tryDirectionBackTiltPlan:
    | function planOk_b = tryDirectionBackTiltPlan()
    | %#codegen
    | %
    | % 自动着陆定向后倾航线规划
    | %
    | % 功能：
    | % 1. 使用与定点盘旋规划相同的高度源；
    | % 2. 当前高度仍需要盘旋降高时，规划失败；
    | % 3. 根据当前水平地速方向确定定向后倾方向；
    | % 4. 水平地速过小时，使用当前偏航角作为后倾方向；
    | % 5. 沿后倾方向向前延伸完整后倾距离；
    | % 6. 后倾过程中保持进入任务时的绝对高度。
    | %
    | % 高度选择：
    | % 1. hagValid_b为true时，使用实测HAG；
    | % 2. hagValid_b为false时，使用当前绝对高度减去Home点地面绝对高度。
    | %
    | % rthPoint_struct.alt_m_f：
    | % Home点地面绝对高度，必须与nav_struct.alt_m_f使用相同高度基准。
    | %
    | % pointLoiterPlanParam：
    | % 1：进入盘旋的高度裕度，m。
    | %
    | % directBwdTiltPlanParam：
    | % 1：完整定向后倾距离，m。
    | 
    | planOk_b = false;
    | 
    | zero_f = single(0.0);
    | radToDeg_f = single(57.29577951308232);
    | 
    | %% 参数读取
    | 
    | loiterEntryMargin_m_f = max(single(pointLoiterPlanParam(1)), zero_f);
    | backTiltTargetHag_m_f = max(single(selectMssnModeParam(2)), zero_f);
    | fullBackTiltDist_m_f = max(single(directBwdTiltPlanParam(1)), zero_f);
    | 
    | currentAlt_m_f = single(nav_struct.alt_m_f);
    | 
    | %% 选择高度源
    | 
    | if nav_struct.hagValid_b
    | 
    |     % HAG有效：使用实测HAG。
    |     hagForPlan_m_f = max(single(nav_struct.hag_m_f), zero_f);
    | 
    | else
    | 
    |     % HAG无效：使用Home点地面绝对高度。
    |     homeGroundAlt_m_f = single(rthPoint_struct.alt_m_f);
    | 
    |     hagForPlan_m_f = currentAlt_m_f - homeGroundAlt_m_f;
    |     hagForPlan_m_f = max(hagForPlan_m_f, zero_f);
    | 
    | end
    | 
    | %% 判断是否允许直接定向后倾
    | 
    | loiterEntryHag_m_f = backTiltTargetHag_m_f + loiterEntryMargin_m_f;
    | 
    | % 当前高度仍高于直接后倾区域，必须先进行盘旋降高。
    | if hagForPlan_m_f > loiterEntryHag_m_f
    |     return;
    | end
    | 
    | %% 计算当前水平地速
    | 
    | velN_mps_f = single(nav_struct.velN_mps_f);
    | velE_mps_f = single(nav_struct.velE_mps_f);
    | 
    | groundSpdSq_m2ps2_f = velN_mps_f * velN_mps_f + velE_mps_f * velE_mps_f;
    | 
    | groundSpd_mps_f = sqrt(max(groundSpdSq_m2ps2_f, zero_f));
    | 
    | %% 计算定向后倾方向
    | 
    | if groundSpd_mps_f >= single(0.1)
    | 
    |     directionBackTiltHdg_deg_f = atan2(velE_mps_f, velN_mps_f) * radToDeg_f;
    | 
    | else
    | 
    |     directionBackTiltHdg_deg_f = single(nav_struct.yaw_deg_f);
    | 
    | end
    | 
    | directionBackTiltHdg_deg_f = cldWrap180(directionBackTiltHdg_deg_f);
    | 
    | %% 计算定向后倾目标位置
    | 
    | referenceLoc_deg_d = [nav_struct.lat_deg_d, nav_struct.lon_deg_d];
    | 
    | backTiltTargetLoc_deg_d = offsetBearing(directionBackTiltHdg_deg_f, fullBackTiltDist_m_f, referenceLoc_deg_d);
    | 
    | %% 生成默认航线
    | 
    | routeTemp_struct = GenerateDefaultRoute();
    | 
    | %% 1号点：后倾起始锚点
    | % yawType_u8，0：航向对准 1：航点指定 2：指向航点
    | routeTemp_struct(1).wpType_u8 = WP_TYPE.FW_LINE_WP;
    | routeTemp_struct(1).lat_deg_d = nav_struct.lat_deg_d;
    | routeTemp_struct(1).lon_deg_d = nav_struct.lon_deg_d;
    | 
    | % 后倾期间保持进入任务时的绝对高度。
    | routeTemp_struct(1).alt_m_f = currentAlt_m_f;
    | 
    | routeTemp_struct(1).spd_mps_f = zero_f;
    | routeTemp_struct(1).radius_m_f = zero_f;
    | routeTemp_struct(1).fastWp_b = false;
    | routeTemp_struct(1).yawType_u8 = uint8(0);
    | routeTemp_struct(1).yaw_deg_f = directionBackTiltHdg_deg_f;
    | routeTemp_struct(1).timeOrCount_u16 = uint16(0);
    | routeTemp_struct(1).arrivalCond_u8 = uint8(0);
    | 
    | %% 2号点：定向后倾目标点
    | 
    | routeTemp_struct(2).wpType_u8 = WP_TYPE.MC_LINE_WP;
    | routeTemp_struct(2).lat_deg_d = backTiltTargetLoc_deg_d(1);
    | routeTemp_struct(2).lon_deg_d = backTiltTargetLoc_deg_d(2);
    | 
    | % 目标点与起始点使用相同绝对高度。
    | routeTemp_struct(2).alt_m_f = currentAlt_m_f;
    | 
    | routeTemp_struct(2).spd_mps_f = zero_f;
    | routeTemp_struct(2).radius_m_f = zero_f;
    | routeTemp_struct(2).fastWp_b = false;
    | routeTemp_struct(2).yawType_u8 = uint8(1);      % 航点指定
    | routeTemp_struct(2).yaw_deg_f = directionBackTiltHdg_deg_f;
    | routeTemp_struct(2).timeOrCount_u16 = uint16(0);
    | routeTemp_struct(2).arrivalCond_u8 = uint8(0);
    | 
    | %% 提交候选航线
    | 
    | candidateRoute_struct = routeTemp_struct;
    | candidateValidWpNum_u8 = uint8(2);
    | candidateRouteUpdate_b = true;
    | 
    | planOk_b = true;
    | 
    | end
  function planOk_b = tryVerticalTakeoffPlan:
    | function planOk_b = tryVerticalTakeoffPlan()
    | %#codegen
    | %
    | % 垂直起飞航线规划
    | %
    | % 功能：
    | % 1. 以进入垂直起飞任务时的当前位置作为起飞锚点；
    | % 2. 在相同经纬度上生成垂直起飞目标航点；
    | % 3. 目标航点高度为当前绝对高度加设定相对起飞高度；
    | % 4. 起飞过程中保持进入任务时的航向；
    | %
    | % 航点定义：
    | % 1号点：起飞锚点，记录任务触发时的位置和高度，不作为执行目标；
    | % 2号点：垂直起飞目标点，是航点更新模块初始执行的当前航点。
    | 
    | routeTemp_struct = GenerateDefaultRoute();
    | 
    | %% 生成起飞锚点
    | 
    | routeTemp_struct(1).wpType_u8 = WP_TYPE.MC_TAKEOFF_WP;
    | routeTemp_struct(1).lat_deg_d = nav_struct.lat_deg_d;
    | routeTemp_struct(1).lon_deg_d = nav_struct.lon_deg_d;
    | routeTemp_struct(1).alt_m_f = nav_struct.alt_m_f;
    | routeTemp_struct(1).spd_mps_f = single(0.0);
    | routeTemp_struct(1).radius_m_f = single(0.0);
    | routeTemp_struct(1).fastWp_b = false;
    | routeTemp_struct(1).yawType_u8 = uint8(0);
    | routeTemp_struct(1).yaw_deg_f = nav_struct.yaw_deg_f;
    | 
    | %% 生成垂直起飞目标点
    | 
    | routeTemp_struct(2) = routeTemp_struct(1);
    | routeTemp_struct(2).alt_m_f = nav_struct.alt_m_f + takeoffRltHgt_m_f;
    | 
    | %% 提交规划结果
    | 
    | candidateRoute_struct = routeTemp_struct;
    | candidateValidWpNum_u8 = uint8(2);
    | candidateRouteUpdate_b = true;
    | planOk_b = candidateRouteUpdate_b;
    | 
    | end
  function planOk_b = tryPointLandPlan:
    | function planOk_b = tryPointLandPlan()
    | %#codegen
    | %
    | % 定点着陆航线规划
    | %
    | % 偏航策略：
    | % 1. 水平刹停方向由predictPointLandStopPoint()根据地速确定；
    | % 2. 定点着陆全过程保持进入规划时的偏航角；
    | % 3. 保证刹停距离预测使用的机体系方向与航线执行一致；
    | % 4. 避免接近刹停点时“指向航点”产生航向跳变。
    | 
    | zero_f = single(0.0);
    | 
    | %% 飞行阶段准入
    | 
    | isMcFlight_b = flightPhase_enum == FLIGHT_PHASE.MC_FLIGHT;
    | 
    | %% 当前运动状态
    | 
    | velN_mps_f = single(nav_struct.velN_mps_f);
    | velE_mps_f = single(nav_struct.velE_mps_f);
    | 
    | groundSpdSq_m2ps2_f = velN_mps_f * velN_mps_f + velE_mps_f * velE_mps_f;
    | 
    | groundSpd_mps_f = sqrt(max(groundSpdSq_m2ps2_f, zero_f));
    | 
    | %% 锁存定点着陆过程偏航角
    | 
    | pointLandYaw_deg_f = cldWrap180(single(nav_struct.yaw_deg_f));
    | 
    | pointLandYawType_u8 = uint8(1);     % 航点指定
    | 
    | %% 预测水平停止位置和垂向停止高度
    | 
    | [stopPos_deg_d, hoverAlt_m_f] = predictPointLandStopPoint(nav_struct, perfParams_struct, pointLandParam, isMcFlight_b);
    | 
    | %% 计算接地点绝对高度
    | 
    | if nav_struct.hagValid_b
    | 
    |     % HAG有效：由当前绝对高度和HAG反算地面绝对高度。
    |     touchdownAlt_m_f = single(nav_struct.alt_m_f) - max(single(nav_struct.hag_m_f), zero_f);
    | 
    | else
    | 
    |     % HAG无效：使用Home点地面绝对高度。
    |     % 必须与nav_struct.alt_m_f使用相同高度基准。
    |     touchdownAlt_m_f = single(rthPoint_struct.alt_m_f);
    | 
    | end
    | 
    | %% 生成默认航线
    | 
    | routeTemp_struct = GenerateDefaultRoute();
    | 
    | %% W1：当前位置锚点
    | 
    | routeTemp_struct(1).wpType_u8 = WP_TYPE.MC_LINE_WP;
    | routeTemp_struct(1).lat_deg_d = nav_struct.lat_deg_d;
    | routeTemp_struct(1).lon_deg_d = nav_struct.lon_deg_d;
    | routeTemp_struct(1).alt_m_f = single(nav_struct.alt_m_f);
    | routeTemp_struct(1).spd_mps_f = groundSpd_mps_f;
    | routeTemp_struct(1).radius_m_f = zero_f;
    | routeTemp_struct(1).fastWp_b = false;
    | 
    | routeTemp_struct(1).yawType_u8 = pointLandYawType_u8;
    | routeTemp_struct(1).yaw_deg_f = pointLandYaw_deg_f;
    | 
    | routeTemp_struct(1).timeOrCount_u16 = uint16(0);
    | routeTemp_struct(1).arrivalCond_u8 = uint8(0);
    | 
    | %% W2：水平、垂向刹停并悬停
    | 
    | routeTemp_struct(2).wpType_u8 = WP_TYPE.MC_LAND_WP;
    | routeTemp_struct(2).lat_deg_d = stopPos_deg_d(1);
    | routeTemp_struct(2).lon_deg_d = stopPos_deg_d(2);
    | routeTemp_struct(2).alt_m_f = hoverAlt_m_f;
    | routeTemp_struct(2).spd_mps_f = zero_f;
    | routeTemp_struct(2).radius_m_f = zero_f;
    | routeTemp_struct(2).fastWp_b = false;
    | 
    | % 保持进入定点着陆时的航向。
    | routeTemp_struct(2).yawType_u8 = pointLandYawType_u8;
    | routeTemp_struct(2).yaw_deg_f = pointLandYaw_deg_f;
    | 
    | routeTemp_struct(2).timeOrCount_u16 = uint16(0);
    | routeTemp_struct(2).arrivalCond_u8 = uint8(0);
    | 
    | %% W3：同一水平位置垂直着陆
    | 
    | if isMcFlight_b
    | 
    |     routeTemp_struct(3).wpType_u8 = WP_TYPE.MC_LAND_WP;
    |     routeTemp_struct(3).lat_deg_d = stopPos_deg_d(1);
    |     routeTemp_struct(3).lon_deg_d = stopPos_deg_d(2);
    |     routeTemp_struct(3).alt_m_f = touchdownAlt_m_f;
    |     routeTemp_struct(3).spd_mps_f = zero_f;
    |     routeTemp_struct(3).radius_m_f = zero_f;
    |     routeTemp_struct(3).fastWp_b = false;
    | 
    |     % 垂直下降过程中导引律中采用的是锁定当前航向角。
    |     routeTemp_struct(3).yawType_u8 = pointLandYawType_u8;
    |     routeTemp_struct(3).yaw_deg_f = pointLandYaw_deg_f;
    | 
    |     routeTemp_struct(3).timeOrCount_u16 = uint16(0);
    |     routeTemp_struct(3).arrivalCond_u8 = uint8(0);
    | 
    |     validWpNumTemp_u8 = uint8(3);
    | 
    | else
    | 
    |     validWpNumTemp_u8 = uint8(2);
    | 
    | end
    | 
    | %% 提交候选规划结果
    | 
    | candidateRoute_struct = routeTemp_struct;
    | candidateValidWpNum_u8 = validWpNumTemp_u8;
    | candidateRouteUpdate_b = true;
    | 
    | planOk_b = true;
    | 
    | end
  function defaultRoute_struct = GenerateDefaultRoute:
    | function defaultRoute_struct = GenerateDefaultRoute()
    | %#codegen
    |     maxNumWp = uint8(30);
    |     wp_struct = struct('wpType_u8',WP_TYPE.INVALID_WP,'lat_deg_d',nav_struct.lat_deg_d,'lon_deg_d',nav_struct.lon_deg_d,...
    |         'alt_m_f',nav_struct.alt_m_f,'spd_mps_f',single(0),'radius_m_f',single(0),'fastWp_b',false,'yawType_u8',uint8(0), ...
    |         'yaw_deg_f',nav_struct.yaw_deg_f,'timeOrCount_u16',uint16(0),'arrivalCond_u8',uint8(0));
    |     defaultRoute_struct = repmat(wp_struct, maxNumWp, 1);
    | end
  function planOk_b = tryAutoLandPlan:
    | function planOk_b = tryAutoLandPlan()
    | %#codegen
    | %
    | % 自动着陆入口预规划。
    | %
    | % 只有一个子规划成功时才返回true，并记录进入哪个子状态。
    | % 所有规划失败时返回false，外层状态不退出。
    | 
    | planOk_b = false;
    | autoLandEntryType_u8 = uint8(0);
    | 
    | %% 固定翼或倾转阶段
    | 
    | if flightPhase_enum == FLIGHT_PHASE.TILT_FLIGHT || ...
    |         flightPhase_enum == FLIGHT_PHASE.FW_FLIGHT
    | 
    |     % 优先尝试定点盘旋降高。
    |     if tryAutoLandPointLoiterPlan()
    | 
    |         autoLandEntryType_u8 = uint8(1);
    |         planOk_b = true;
    |         return;
    | 
    |     end
    | 
    |     % 不需要盘旋或盘旋规划不成立时，尝试定向后倾。
    |     %
    |     % tryDirectionBackTiltPlan内部必须包含互补高度判断：
    |     % 高度较高且应先盘旋时，不允许直接后倾。
    |     if tryDirectionBackTiltPlan()
    | 
    |         autoLandEntryType_u8 = uint8(2);
    |         planOk_b = true;
    |         return;
    | 
    |     end
    | 
    | %% 旋翼飞行或地面阶段
    | 
    | elseif flightPhase_enum == FLIGHT_PHASE.MC_FLIGHT || ...
    |         flightPhase_enum == FLIGHT_PHASE.MC_GROUND
    | 
    |     if tryPointLandPlan()
    | 
    |         autoLandEntryType_u8 = uint8(3);
    |         planOk_b = true;
    |         return;
    | 
    |     end
    | 
    | end
    | 
    | end
